simulink subsystem "VehSpdRef_HighSpeed_refsub"  (R2025a)
settings: Solver=VariableStepAuto  StartTime=0.0  StopTime=10.0  RelTol=1e-3
libraries: simulink x1
settings Model: Creator=isaacito  LastModifiedBy=isaacito
settings OptimizationCC: ReuseModelBlockBuffer=off
settings RTWCC: GPUComputeCapability=3.5

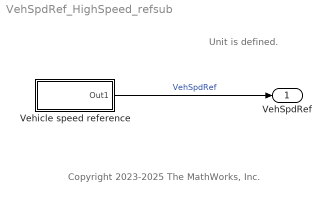
== system VehSpdRef_HighSpeed_refsub ==
  note: Unit is defined.
  note: Copyright 2023-2025 The MathWorks, Inc.
  Vehicle speed reference : Subsystem  mask(Trace Generator){yScale=1, tScale=1, randomSeed=6, interpolationStepSize=0.5, tInitialFlatLength=10, yInitialValue=0, numTransitions=10, transitionRange=[5 10], flatRange=[5 10], yRange=[60 100], tFinalTransitionDuration=15, tFinalFlatDuration=10, yFinalValue=0}
      mask prompts: yScale "Data value scaler"; tScale "Time scaler"; randomSeed "Random seed"; interpolationStepSize "Interpolation step [s]"; tInitialFlatLength "Initial constant duration"; yInitialValue "Initial data value"; numTransitions "Number of transitions"; transitionRange "Range of transition duration"; flatRange "Range of constant duration"; yRange "Range of data value"; tFinalTransitionDuration "Final transition duration"; tFinalFlatDuration "Final constant duration"; yFinalValue "Final data value"
      mask help: This block generates a smooth signal consisting of flat segments.
      mask init:
      | xydata = SignalDesignUtility.buildXYData( ...
      |   RandomSeed = randomSeed, ...
      |   XScale = tScale, ...
      |   YScale = yScale, ...
      |   XInitialFlatLength = tInitialFlatLength, ...
      |   YInitialValue = yInitialValue, ...
      |   NumTransitions  = numTransitions, ...
      |   TransitionRange = transitionRange, ...
      |   FlatRange = flatRange, ...
      |   YRange = yRange, ...
      |   XFinalTransitionLength = tFinalTransitionDuration, ...
      |   XFinalFlatLength = tFinalFlatDuration, ...
      |   YFinalValue = yFinalValue );
      | 
      | sig = SignalDesigner("ContinuousMultiStep");
      | sig.XYData = xydata;
      | sig.DeltaX = interpolationStepSize;
      | 
      | update(sig)
      mask DialogControl Container3 Prompt: Advanced
      mask DialogControl Control3 Prompt: horizontal spacer 1
      mask DialogControl Control4 Prompt: horizontal spacer 2
      mask DialogControl Control5 Prompt: horizontal spacer 3
      mask DialogControl PlotButton Prompt: Plot
      mask DialogControl PlotButton Callback: SignalSourceBlockCallback.plotTraceGenerator(gcb);
      mask Display: disp("Trace" + newline + "Generator")
  VehSpdRef : Outport  Unit=km/h
      settings: AttributesFormatString=%<Unit>
  wires:
  Vehicle speed reference/1(Out1) -> VehSpdRef/1  "VehSpdRef"

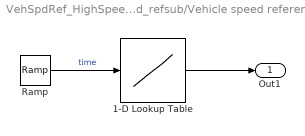
== system VehSpdRef_HighSpeed_refsub/Vehicle speed reference ==
  1-D Lookup Table : Lookup_n-D  NumberOfTableDimensions=1  BreakpointsForDimension1=sig.Data.X  Table=sig.Data.Y  InternalRulePriority=Speed  RndMeth=Simplest
  Ramp : simulink/Sources/Ramp  slope=1  start=0  InitialOutput=0
      settings: AttributesFormatString=|
      | Slope: %<slope>
      | Start time: %<start>
      | Initial output: %<InitialOutput>
  Out1 : Outport
  wires:
  1-D Lookup Table/1 -> Out1/1
  Ramp/1 -> 1-D Lookup Table/1  "time"
